simulink model "commhdlQPSKTxRx"  (R2025b)
settings: Solver=FixedStepDiscrete  StartTime=0.0  StopTime=stopTime  RelTol=1e-3
PostLoadFcn:
  | hScopeConfig = get_param([gcs '/Receiver/QPSK Rx/Frequency and Time Synchronizer/Symbol Synchronizer/No HDL/QPSK Receiver Eye Diagram'],'ScopeConfiguration');
  | 
  | hScopeConfig.OpenAtSimulationStart = false;
  | hScopeConfig.Visible = false;
  | SamplesPerSymbol = 4;
  | %UpsamplesRx = 1;
  | clear hScopeConfig
InitFcn:
  | commhdlQPSKTxRxModelInit;
  | % Rate bridge: ADRV9002/Jupiter radio runs at 15.36 MHz = 2x the 7.68 MHz
  | % (4 samples/symbol @ Rsym=1.92 MHz) the QPSK Rx requires. The deployed
  | % Receiver must downsample the ADC stream by 2. UpsamplesRx=1 fed the QPSK
  | % Rx 8 sps (2x-upsampled) and broke symbol sync / the loopback bit check.
  | UpsamplesRx = 1;   %% T8 RATE FIX: rail 15.36e6 == ADC bus rate,
  | %% no ingress decimation (was 2 when the rail sat on the 7.68e6 rung)
  | UpsamplesTx = 1;
  | clear simTimingOffset;
StopFcn:
  | if exist('simTimingOffset','var')
  |   disp('Simulation completed');
  |   %QPSKTxRxVerification;
  | end
undefined symbols (not defined in the file or in its folder): Add, Config, fsym, randsrc, RandStream, Rsym, Shift
libraries: hdlsllib x76, simulink x21, dspsigops x19, dsphdlfiltering2 x3, dsphdlsigops2 x2, dsphdlmathfun2 x2, commdigbbndpm3 x2, commchan3 x1, commrflib2 x1
(part 3 of 4)

== system commhdlQPSKTxRx/Receiver/QPSK Rx/Frequency and Time Synchronizer/Phase Ambiguity Estimation and Correction/Phase Ambiguity Estimator ==
  dataIn : Inport
  syncPulse : Inport  Port=2
  validIn : Inport  Port=3
  Compare To Constant : simulink/Logic and Bit Operations/Compare To Constant  relop===  const=7  OutDataTypeStr=boolean
  Delay{1..3,8} (4 alike) : Delay  DelayLength=1
  Delay{4..7,9..11} (7 alike) : Delay
  Direct Lookup Table (n-D) : LookupNDDirect  NumberOfTableDimensions=1  Table=fi(preambleSymbols(3+1:3+8),1,16)  DiagnosticForOutOfRangeInput=Error
  HDL Counter : hdlsllib/Sources/HDL Counter  CountType=Count limited  CountInit=0  CountStep=1  CountMax=8-1  CountFromType=Initial value  CountFrom=0  CountResetPort=on  CountLoadPort=off  CountEnbPort=on  CountDirPort=off  CountHitOutputPort=off  CountDataType=Unsigned  CountWordLen=3  CountFracLen=0  CountSampTime=1
  Logical Operator : Logic  IconShape=distinctive  AllPortsSameDT=off  OutDataTypeStr=boolean
  Math Function : Math  Operator=conj  SignedPower=on  RndMeth=Zero
  Product : Product
  Subsystem : Subsystem
  Subsystem1 : Subsystem
  endOut : Outport
  estOut : Outport  Port=2
  validOut : Outport  Port=3
  wires:
  Compare To Constant/1 -> Logical Operator/2
  Subsystem/1(Out2) -> Subsystem1/1(In1), HDL Counter/1
  Direct Lookup Table (n-D)/1 -> Math Function/1
  Math Function/1 -> Delay4/1
  Product/1 -> Delay9/1
  Delay8/1 -> Direct Lookup Table (n-D)/1
  Delay1/1 -> Delay5/1
  Delay2/1 -> Delay6/1
  Delay3/1 -> Delay7/1
  Delay4/1 -> Product/2
  Delay5/1 -> Product/1
  Delay6/1 -> Delay10/1
  Delay7/1 -> Delay11/1
  Delay9/1 -> estOut/1
  Delay10/1 -> validOut/1
  Delay11/1 -> endOut/1
  dataIn/1 -> Delay1/1
  HDL Counter/1 -> Delay8/1, Compare To Constant/1
  Subsystem1/1(validOut) -> Delay2/1, Logical Operator/1, HDL Counter/2
  Logical Operator/1 -> Delay3/1, Subsystem/2(H)
  syncPulse/1 -> Subsystem/1(L)
  validIn/1 -> Subsystem1/2(validIn)

== system commhdlQPSKTxRx/Receiver/QPSK Rx/Frequency and Time Synchronizer/Preamble Detector/Correlator ==
  dataIn : Inport
  validIn : Inport  Port=2
  Complex to Real-Imag : ComplexToRealImag  Output=Real
  Delay{1..6} (6 alike) : Delay  DelayLength=1
  Delay7 : Delay  DelayLength=4
  Delay8 : Delay  DelayLength=4
  Discrete FIR Filter : dsphdlfiltering2/Discrete FIR Filter  NumeratorSource=Property  Numerator=rxPreambleMFCoeffs  NumeratorPrototype=[]  FilterStructure=Direct form systolic  SerializationOption=Minimum number of cycles between valid input samples  NumCycles=2  NumberOfMultipliers=2  SimulateUsing=Code generation  roundingMode=Floor  overflowMode=off  CoefficientsDataTypeStr=Inherit: Same word length as input  OutputDataTypeStr=Inherit: Same word length as input  ResetInputPort=off  HDLGlobalReset=off  CoeffMultiplier=Multiplier  UseMultForPow2Coeff=on  FrameInputSymmOptim=off
  Magnitude Squared : Subsystem
  Magnitude Squared and Moving Sum : Subsystem
  ThresholdLimiter : MATLAB Function  TreatAsAtomicUnit=on
  dataOut : Outport
  threshold : Outport  Port=2
  validOut : Outport  Port=3
  wires:
  Discrete FIR Filter/2 -> Delay1/1
  validIn/1 -> Magnitude Squared and Moving Sum/2(validIn), Discrete FIR Filter/2
  Discrete FIR Filter/1 -> Delay6/1
  Delay1/1 -> Delay7/1
  Delay3/1 -> validOut/1
  dataIn/1 -> Magnitude Squared and Moving Sum/1(scaled1), Discrete FIR Filter/1
  Delay4/1 -> ThresholdLimiter/1(x)
  Delay2/1 -> dataOut/1
  Delay5/1 -> threshold/1
  Magnitude Squared and Moving Sum/1(E1) -> Delay4/1
  Delay6/1 -> Magnitude Squared/1(In1)
  Magnitude Squared/1(Out1) -> Complex to Real-Imag/1
  ThresholdLimiter/1(y) -> Delay8/1
  Delay7/1 -> Delay3/1
  Delay8/1 -> Delay5/1
  Complex to Real-Imag/1 -> Delay2/1

== system commhdlQPSKTxRx/Receiver/QPSK Rx/Frequency and Time Synchronizer/Preamble Detector/FIFO ==
  in : Inport
  push : Inport  Port=2
  pop : Inport  Port=3
  reset : Inport  Port=4
  Delay1 : Delay  DelayLength=1
  Pop Counter : hdlsllib/Sources/HDL Counter  CountType=Count limited  CountInit=0  CountStep=1  CountMax=fifoSize -1  CountFromType=Initial value  CountFrom=0  CountResetPort=on  CountLoadPort=off  CountEnbPort=on  CountDirPort=off  CountHitOutputPort=off  CountDataType=Unsigned  CountWordLen=nextpow2(fifoSize)  CountFracLen=0  CountSampTime=1
  Push Counter : hdlsllib/Sources/HDL Counter  CountType=Count limited  CountInit=0  CountStep=1  CountMax=fifoSize -1  CountFromType=Initial value  CountFrom=0  CountResetPort=on  CountLoadPort=off  CountEnbPort=on  CountDirPort=off  CountHitOutputPort=off  CountDataType=Unsigned  CountWordLen=nextpow2(fifoSize)  CountFracLen=0  CountSampTime=1
  Simple Dual Port RAM : hdlsllib/HDL RAMs/Simple Dual Port RAM  ram_size=nextpow2(fifoSize)
  Validate Input Push Pop : Subsystem
  out : Outport
  numEntries : Outport  Port=2
  validPop : Outport  Port=3
  wires:
  Delay1/1 -> Push Counter/1, Pop Counter/1
  in/1 -> Simple Dual Port RAM/1
  reset/1 -> Validate Input Push Pop/1(rst), Delay1/1
  Validate Input Push Pop/2(valid pop) -> Pop Counter/2, validPop/1
  Validate Input Push Pop/1(valid push) -> Push Counter/2, Simple Dual Port RAM/3
  pop/1 -> Validate Input Push Pop/3(pop)
  push/1 -> Validate Input Push Pop/2(push)
  Pop Counter/1 -> Simple Dual Port RAM/4
  Push Counter/1 -> Simple Dual Port RAM/2
  Simple Dual Port RAM/1 -> out/1
  Validate Input Push Pop/3(numEntries) -> numEntries/1

== system commhdlQPSKTxRx/Receiver/QPSK Rx/Frequency and Time Synchronizer/Preamble Detector/No HDL ==
  In1 : Inport
  In2 : Inport  Port=2
  Enable : EnablePort
  Correlation Time Scope : Scope  NumInputPorts=2
      settings: TimeUnits=Metric (based on Time Span)  Title=Time Plot of Preamble Detection  ActiveDisplayYMinimum=-0.38501295493915666  ActiveDisplayYMaximum=3.4651165944524109  YLabel=Amplitude
  Data Type Conversion : DataTypeConversion  OutDataTypeStr=double  SaturateOnIntegerOverflow=off  RndMeth=Floor
  Data Type Conversion1 : DataTypeConversion  OutDataTypeStr=double  SaturateOnIntegerOverflow=off  RndMeth=Floor
  To Workspace : ToWorkspace  VariableName=simPeakFind  SampleTime=-1
      settings: Save2DSignal=2-D array (concatenate along first dimension)
  wires:
  Data Type Conversion1/1 -> Correlation Time Scope/2  "Threshold"
  In2/1 -> Data Type Conversion1/1
  Data Type Conversion/1 -> To Workspace/1, Correlation Time Scope/1  "Correlation Value"
  In1/1 -> Data Type Conversion/1

== system commhdlQPSKTxRx/Receiver/QPSK Rx/Frequency and Time Synchronizer/Preamble Detector/Peak Search ==
  note: peak picker
  corr : Inport
  thresholdExceeded : Inport  Port=2
  validIn : Inport  Port=3
  Compare To Constant : simulink/Logic and Bit Operations/Compare To Constant  relop===  const=samplesPerFrame1x - 1  OutDataTypeStr=boolean
  Logical Operator : Logic  IconShape=distinctive  AllPortsSameDT=off  OutDataTypeStr=boolean
  Logical Operator4 : Logic  IconShape=distinctive  AllPortsSameDT=off  OutDataTypeStr=boolean
  Relational Operator : RelationalOperator  Operator=>  OutDataTypeStr=boolean  InputSameDT=off
  Terminator : Terminator
  Unit Delay Enabled Synchronous : hdlsllib/Discrete/Unit Delay Enabled Synchronous  InitialCondition=0.0  SampleTime=-1
  Unit Delay Enabled Synchronous1 : hdlsllib/Discrete/Unit Delay Enabled Synchronous  InitialCondition=0.0  SampleTime=-1
  Unit Delay Enabled Resettable Synchronous : hdlsllib/Discrete/Unit Delay Enabled Resettable Synchronous  InitialCondition=0.0  SampleTime=-1
  Unit Delay Enabled Resettable Synchronous1 : hdlsllib/Discrete/Unit Delay Enabled Resettable Synchronous  InitialCondition=0.0  SampleTime=-1
  timing Reference : hdlsllib/Sources/HDL Counter  CountType=Count limited  CountInit=0  CountStep=1  CountMax=samplesPerFrame1x - 1  CountFromType=Initial value  CountFrom=0  CountResetPort=off  CountLoadPort=off  CountEnbPort=on  CountDirPort=off  CountHitOutputPort=off  CountDataType=Unsigned  CountWordLen=nextpow2(samplesPerFrame1x - 1)  CountFracLen=0  CountSampTime=1
  timing Reference Long : hdlsllib/Sources/HDL Counter  CountType=Free running  CountInit=0  CountStep=1  CountMax=samplesPerFrame1x - 1  CountFromType=Initial value  CountFrom=0  CountResetPort=off  CountLoadPort=off  CountEnbPort=on  CountDirPort=off  CountHitOutputPort=off  CountDataType=Unsigned  CountWordLen=32  CountFracLen=0  CountSampTime=1
  timingOffset : Outport
  done : Outport  Port=2
  success : Outport  Port=3
  wires:
  validIn/1 -> Logical Operator/1, timing Reference/1, timing Reference Long/1
  timing Reference Long/1 -> Unit Delay Enabled Synchronous1/1
  timing Reference/1 -> Unit Delay Enabled Synchronous/1, Compare To Constant/1
  thresholdExceeded/1 -> Unit Delay Enabled Resettable Synchronous1/2, Unit Delay Enabled Resettable Synchronous1/1, Logical Operator4/2
  corr/1 -> Unit Delay Enabled Resettable Synchronous/1, Relational Operator/1
  Compare To Constant/1 -> Logical Operator/2
  Logical Operator/1 -> Unit Delay Enabled Resettable Synchronous1/3, done/1, Unit Delay Enabled Resettable Synchronous/3
  Relational Operator/1 -> Logical Operator4/1
  Unit Delay Enabled Resettable Synchronous/1 -> Relational Operator/2
  Unit Delay Enabled Resettable Synchronous1/1 -> success/1
  Logical Operator4/1 -> Unit Delay Enabled Synchronous/2, Unit Delay Enabled Synchronous1/2, Unit Delay Enabled Resettable Synchronous/2
  Unit Delay Enabled Synchronous/1 -> timingOffset/1
  Unit Delay Enabled Synchronous1/1 -> Terminator/1

== system commhdlQPSKTxRx/Receiver/QPSK Rx/Frequency and Time Synchronizer/Preamble Detector/Timing Adjust ==
  timingOffset : Inport
  timingOffsetValid : Inport  Port=2
  dataIn : Inport  Port=3
  validIn : Inport  Port=4
  Delay{,1..4} (5 alike) : Delay  DelayLength=1
  Logical Operator : Logic  AllPortsSameDT=off  OutDataTypeStr=boolean
  Logical Operator1 : Logic  Operator=NOT  AllPortsSameDT=off  OutDataTypeStr=boolean
  Logical Operator2 : Logic  Inputs=3  AllPortsSameDT=off  OutDataTypeStr=boolean
  No HDL : Subsystem
  Relational Operator : RelationalOperator  Operator===  OutDataTypeStr=boolean  InputSameDT=off
  State Register : hdlsllib/Discrete/Unit Delay Enabled Resettable Synchronous  InitialCondition=0.0  SampleTime=-1
  Unit Delay Enabled Synchronous3 : hdlsllib/Discrete/Unit Delay Enabled Synchronous  InitialCondition=0.0  SampleTime=-1
  timing Reference : hdlsllib/Sources/HDL Counter  CountType=Count limited  CountInit=0  CountStep=1  CountMax=searchSamples - 1  CountFromType=Initial value  CountFrom=0  CountResetPort=off  CountLoadPort=off  CountEnbPort=on  CountDirPort=off  CountHitOutputPort=off  CountDataType=Unsigned  CountWordLen=nextpow2(searchSamples - 1)  CountFracLen=0  CountSampTime=1
  dataOut : Outport
  validOut : Outport  Port=2
  SyncPulse : Outport  Port=3
  wires:
  Delay4/1 -> dataOut/1
  Delay3/1 -> validOut/1
  timingOffset/1 -> Unit Delay Enabled Synchronous3/1
  Unit Delay Enabled Synchronous3/1 -> Relational Operator/2
  Delay/1 -> SyncPulse/1
  validIn/1 -> timing Reference/1, Logical Operator2/1, No HDL/1(validIn), Delay3/1
  State Register/1 -> Logical Operator2/3, Delay1/1
  Logical Operator1/1 -> Logical Operator/2
  Relational Operator/1 -> Logical Operator2/2
  Logical Operator2/1 -> No HDL/3(syncPulse), Delay/1, Delay2/1
  Delay2/1 -> State Register/3
  Logical Operator/1 -> State Register/1, State Register/2, Unit Delay Enabled Synchronous3/2
  timing Reference/1 -> No HDL/2(timingOffset), Relational Operator/1
  timingOffsetValid/1 -> Logical Operator/1
  Delay1/1 -> Logical Operator1/1
  dataIn/1 -> Delay4/1

== system commhdlQPSKTxRx/Receiver/QPSK Rx/Frequency and Time Synchronizer/Symbol Synchronizer/Gardner TED ==
  data : Inport
  strobe : Inport  Port=2
  Constant : Constant  Value=0  OutDataTypeStr=Inherit: Inherit via back propagation  SampleTime=1/(Rsym*SamplesPerSymbol)
  Delay10 : Delay  DelayLength=4
  GTED : Subsystem
  Switch : Switch  Criteria=u2 ~= 0  InputSameDT=off
  e : Outport  VectorParamsAs1DForOutWhenUnconnected=off
  wires:
  Constant/1 -> Switch/3
  Switch/1 -> e/1
  strobe/1 -> Delay10/1
  data/1 -> GTED/1(In1)
  GTED/1(Out1) -> Switch/1
  Delay10/1 -> Switch/2

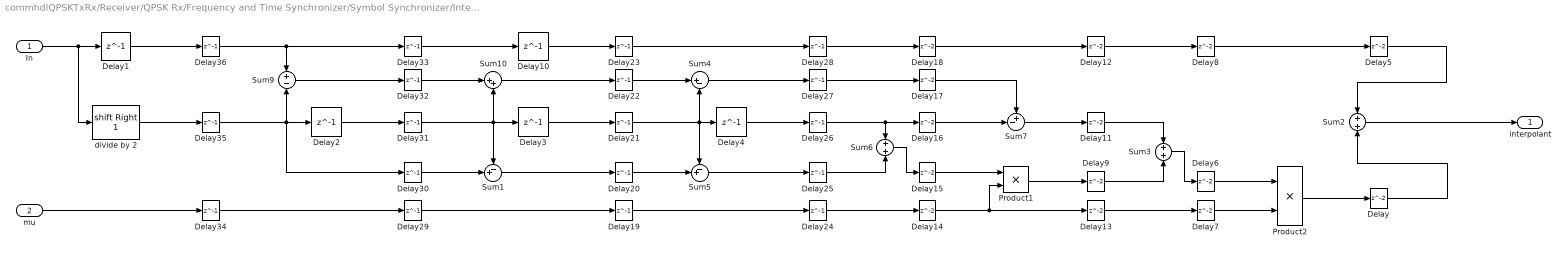
== system commhdlQPSKTxRx/Receiver/QPSK Rx/Frequency and Time Synchronizer/Symbol Synchronizer/Interpolation Filter ==
  In : Inport
  mu : Inport  Port=2
  Delay{,5..9,11..18} (14 alike) : Delay
  Delay{1..4,10} (5 alike) : Delay  DelayLength=1  InitialCondition=0
  Delay{19..36} (18 alike) : Delay  DelayLength=1
  Product1 : Product  OutDataTypeStr=fixdt(1,16,10)  RndMeth=Zero
  Product2 : Product  RndMeth=Zero  OutDataTypeStr=Inherit: Same as first input
  Sum1 : Sum  Inputs=-+|
  Sum10 : Sum  Inputs=|++
  Sum2 : Sum  Inputs=+|+
  Sum3 : Sum  Inputs=+|+  OutDataTypeStr=fixdt(1,16,10)
  Sum4 : Sum  Inputs=|+-
  Sum5 : Sum  Inputs=-+|
  Sum6 : Sum  Inputs=+|+  OutDataTypeStr=fixdt(1,16,11)  SaturateOnIntegerOverflow=on
  Sum7 : Sum  Inputs=+-|  OutDataTypeStr=fixdt(1,16,10)
  Sum9 : Sum  Inputs=+-
  divide by 2 : ArithShift  BitShiftNumber=1  BitShiftDirection=Right
  interpolant : Outport
  wires:
  Sum9/1 -> Delay32/1
  In/1 -> divide by 2/1, Delay1/1
  Sum2/1 -> interpolant/1
  Sum7/1 -> Delay11/1
  Product1/1 -> Delay9/1
  Product2/1 -> Delay/1
  Sum3/1 -> Delay6/1
  Sum1/1 -> Delay20/1
  Delay3/1 -> Delay21/1
  Sum10/1 -> Delay22/1
  Delay2/1 -> Delay31/1
  Delay1/1 -> Delay36/1
  divide by 2/1 -> Delay35/1
  Delay/1 -> Sum2/2
  Delay5/1 -> Sum2/1
  Delay6/1 -> Product2/1
  Delay7/1 -> Product2/2
  Delay8/1 -> Delay5/1
  Delay9/1 -> Sum3/2
  Delay11/1 -> Sum3/1
  Delay12/1 -> Delay8/1
  Delay13/1 -> Delay7/1
  Delay14/1 -> Delay13/1, Product1/2
  Delay15/1 -> Product1/1
  Delay16/1 -> Sum7/2
  Delay17/1 -> Sum7/1
  Delay18/1 -> Delay12/1
  mu/1 -> Delay34/1
  Sum5/1 -> Delay25/1
  Delay4/1 -> Delay26/1
  Sum4/1 -> Delay27/1
  Delay10/1 -> Delay23/1
  Delay24/1 -> Delay14/1
  Sum6/1 -> Delay15/1
  Delay26/1 -> Delay16/1, Sum6/1
  Delay27/1 -> Delay17/1
  Delay28/1 -> Delay18/1
  Delay25/1 -> Sum6/2
  Delay19/1 -> Delay24/1
  Delay20/1 -> Sum5/2
  Delay21/1 -> Sum4/2, Sum5/1, Delay4/1
  Delay22/1 -> Sum4/1
  Delay23/1 -> Delay28/1
  Delay29/1 -> Delay19/1
  Delay30/1 -> Sum1/2
  Delay31/1 -> Sum1/1, Sum10/2, Delay3/1
  Delay32/1 -> Sum10/1
  Delay33/1 -> Delay10/1
  Delay34/1 -> Delay29/1
  Delay35/1 -> Delay30/1, Delay2/1, Sum9/2
  Delay36/1 -> Delay33/1, Sum9/1

== system commhdlQPSKTxRx/Receiver/QPSK Rx/Frequency and Time Synchronizer/Symbol Synchronizer/Loop Filter ==
  note: Proportional-Plus-Integrator Loop Filter,
      | Infinite DC Response to guarantee convergence
  e : Inport
  Add : Sum
  Add2 : Sum  Inputs=|++  OutDataTypeStr=Inherit: Same as first input
  Data Type Conversion17 : DataTypeConversion  OutDataTypeStr=fixdt(1,11,10)  RndMeth=Floor
  Delay : Delay  DelayLength=1
  Delay1 : Delay  DelayLength=1  InitialCondition=0
  Delay2 : Delay  InitialCondition=0
  Delay3 : Delay  InitialCondition=0
  Delay4 : Delay  DelayLength=1  InitialCondition=0
  Delay5 : Delay  InitialCondition=0
  Delay6 : Delay  DelayLength=1
  IntegClamp : Saturate  UpperLimit=0.06  LowerLimit=-0.06
  K1 : Gain  Gain=fi(SSLoopFilterPropGain,1,24,24)  ParamDataTypeStr=Inherit: Inherit from 'Gain'  OutDataTypeStr=fixdt(1,30,23)
  K2 : Gain  Gain=fi(SSLoopFilterIntegGain,1,24,24)  ParamDataTypeStr=Inherit: Inherit from 'Gain'  OutDataTypeStr=fixdt(1,30,23)
  v : Outport
  wires:
  Delay/1 -> Add2/2
  Delay5/1 -> Delay6/1
  Delay3/1 -> Delay1/1
  e/1 -> Delay2/1
  Add/1 -> Data Type Conversion17/1
  Delay1/1 -> Add/1
  Delay4/1 -> Add/2
  Delay2/1 -> K1/1, K2/1
  Data Type Conversion17/1 -> v/1
  K2/1 -> Delay5/1
  K1/1 -> Delay3/1
  Delay6/1 -> Add2/1
  Add2/1 -> IntegClamp/1
  IntegClamp/1 -> Delay/1, Delay4/1

== system commhdlQPSKTxRx/Receiver/QPSK Rx/Frequency and Time Synchronizer/Symbol Synchronizer/No HDL ==
  data : Inport
  valid : Inport  Port=2
  Data Type Conversion : DataTypeConversion  OutDataTypeStr=double  SaturateOnIntegerOverflow=off  RndMeth=Floor
  No HDL : Subsystem
  QPSK Receiver Eye Diagram : EyeDiagramBlock  WindowPosition=[403.000000,370.000000,417.000000,506.000000,]  ScopeFrameLocation=window  SamplesPerSymbol=SamplesPerSymbol  SymbolsPerTrace=1  Title=RRC Matched Filtered Output  YLimits=[-1.1602,1.2629]
      settings: OpenAtSimulationStart=off
  Unit Delay Enabled Synchronous : hdlsllib/Discrete/Unit Delay Enabled Synchronous  InitialCondition=0.0  SampleTime=-1
  wires:
  data/1 -> No HDL/1(data), Unit Delay Enabled Synchronous/1
  Unit Delay Enabled Synchronous/1 -> Data Type Conversion/1
  valid/1 -> Unit Delay Enabled Synchronous/2, No HDL/Enable
  Data Type Conversion/1 -> QPSK Receiver Eye Diagram/1

== system commhdlQPSKTxRx/Receiver/QPSK Rx/Frequency and Time Synchronizer/Symbol Synchronizer/Rate Handle ==
  dataIn : Inport
  strobe : Inport  Port=2
  validIn : Inport  Port=3
  Compare To Constant : simulink/Logic and Bit Operations/Compare To Constant  relop===  const=0  OutDataTypeStr=boolean
  Constant : Constant  Value=false  SampleTime=-1
  FIFO : Subsystem  mask{fifoSize=32, pushFullDiag=Error, popEmptyDiag=Ignore}
      mask prompts: fifoSize "FIFO size:"; pushFullDiag "Push full FIFO:"; popEmptyDiag "Pop empty FIFO:"
      mask TypeOptions pushFullDiag: Ignore | Warning | Error
      mask TypeOptions popEmptyDiag: Ignore | Warning | Error
  HDL Counter : hdlsllib/Sources/HDL Counter  CountType=Count limited  CountInit=0  CountStep=1  CountMax=SamplesPerSymbol - 1  CountFromType=Initial value  CountFrom=0  CountResetPort=off  CountLoadPort=off  CountEnbPort=on  CountDirPort=off  CountHitOutputPort=off  CountDataType=Unsigned  CountWordLen=nextpow2(SamplesPerSymbol - 1)  CountFracLen=0  CountSampTime=1
  Logical Operator : Logic  AllPortsSameDT=off  OutDataTypeStr=boolean
  Terminator : Terminator
  dataOut : Outport
  validOut : Outport  Port=2
  wires:
  strobe/1 -> FIFO/2(push)
  dataIn/1 -> FIFO/1(in)
  validIn/1 -> Logical Operator/1, HDL Counter/1
  HDL Counter/1 -> Compare To Constant/1
  Compare To Constant/1 -> Logical Operator/2
  Logical Operator/1 -> FIFO/3(pop)
  FIFO/1(out) -> dataOut/1
  FIFO/3(validPop) -> validOut/1
  FIFO/2(numEntries) -> Terminator/1
  Constant/1 -> FIFO/4(reset)

== system commhdlQPSKTxRx/Transmitter/QPSK Tx/Bit Packetizer/Data Bits FIFO/No HDL ==
  push : Inport
  pop : Inport  Port=2
  MATLAB Function : MATLAB Function  TreatAsAtomicUnit=on
  No HDL : Subsystem
  wires:
  push/1 -> MATLAB Function/1(wr), No HDL/1(push)
  pop/1 -> MATLAB Function/2(rd), No HDL/5(pop)
  MATLAB Function/2(ncount) -> No HDL/3(ncount)
  MATLAB Function/1(full) -> No HDL/2(full)
  MATLAB Function/3(empty) -> No HDL/4(empty)

== system commhdlQPSKTxRx/Transmitter/QPSK Tx/Bit Packetizer/Preamble Bits Generator/Preamble Bits Store ==
  note: The Preamble is padded with zeros in the LUT such that
      | the length is the 2^nextpow2(length(Preamble)) for
      | efficient resource mapping to RAM
  actualPreamble : Inport
  sampleCount : Inport  Port=2
  Constant : Constant  OutDataTypeStr=boolean  SampleTime=1/(Rsym*SamplesPerSymbol)
  Extract Bits : simulink/Logic and Bit Operations/Extract Bits  bitsToExtract=Range of bits  numBits=8  bitIdxRange=[0 nextpow2(length(Preamble))-1]  outScalingMode=Treat bit field as an integer
  Preamble : LookupNDDirect  NumberOfTableDimensions=1  Table=[Preamble;false(32-length(Preamble),1)]  DiagnosticForOutOfRangeInput=Error
  Switch : Switch  Criteria=u2 ~= 0  Threshold=1  SaturateOnIntegerOverflow=off  InputSameDT=off
  preamble : Outport
  wires:
  Switch/1 -> preamble/1
  Constant/1 -> Switch/3
  Extract Bits/1 -> Preamble/1
  Preamble/1 -> Switch/1
  sampleCount/1 -> Extract Bits/1
  actualPreamble/1 -> Switch/2

== system commhdlQPSKTxRx/Receiver/QPSK Rx/Frequency and Time Synchronizer/Coarse Frequency Compensator/Coarse Frequency Estimator/Extract Frequency ==
  datain : Inport
  validIn : Inport  Port=2
  Complex to Magnitude-Angle HDL Optimized : dsphdlmathfun2/Complex to Magnitude-Angle  NumIterationsSource=Auto  NumIterations=10  OutputFormat=Angle  AngleFormat=Normalized  ScaleOutput=on  ScalingMethod=Shift-Add  SimulateUsing=Code generation
  Delay{1..4} (4 alike) : Delay  DelayLength=1
  Gain : Gain  Gain=1/2  ParamDataTypeStr=fixdt(0,1,1)  OutDataTypeStr=Inherit: Same as input
  Unit Delay Enabled Synchronous : hdlsllib/Discrete/Unit Delay Enabled Synchronous  InitialCondition=0.0  SampleTime=-1
  normFreqOut : Outport
  wires:
  Unit Delay Enabled Synchronous/1 -> Delay2/1
  Complex to Magnitude-Angle HDL Optimized/2 -> Unit Delay Enabled Synchronous/2
  datain/1 -> Delay1/1
  Gain/1 -> Delay3/1
  Delay1/1 -> Complex to Magnitude-Angle HDL Optimized/1
  Delay2/1 -> Gain/1
  Delay3/1 -> normFreqOut/1
  validIn/1 -> Delay4/1
  Delay4/1 -> Complex to Magnitude-Angle HDL Optimized/2
  Complex to Magnitude-Angle HDL Optimized/1 -> Unit Delay Enabled Synchronous/1

== system commhdlQPSKTxRx/Receiver/QPSK Rx/Frequency and Time Synchronizer/Coarse Frequency Compensator/Coarse Frequency Estimator/Integrator ==
  note: store the value in the Reg before reset
  dataIn : Inport
  validIn : Inport  Port=2
  Add1 : Sum  Inputs=|++  OutDataTypeStr=Inherit: Same as first input
  Delay : Delay  DelayLength=1
  Delay1 : Delay  DelayLength=1
  Delay2 : Delay  DelayLength=1
  Integ Reg : hdlsllib/Discrete/Unit Delay Enabled Resettable Synchronous  InitialCondition=0.0  SampleTime=-1
  Reset Generator : Subsystem
  Store Reg : hdlsllib/Discrete/Unit Delay Enabled Synchronous  InitialCondition=0.0  SampleTime=-1
  IntegOut : Outport
  IntegValid : Outport  Port=2
  wires:
  Add1/1 -> Integ Reg/1
  Integ Reg/1 -> Store Reg/1, Add1/2
  validIn/1 -> Delay2/1, Reset Generator/1(validIn)
  dataIn/1 -> Delay1/1
  Delay1/1 -> Add1/1
  Delay/1 -> IntegValid/1
  Store Reg/1 -> IntegOut/1
  Reset Generator/1(reset) -> Delay/1, Store Reg/2, Integ Reg/3
  Delay2/1 -> Integ Reg/2

== system commhdlQPSKTxRx/Receiver/QPSK Rx/Frequency and Time Synchronizer/Phase Ambiguity Estimation and Correction/Phase Ambiguity Corrector/Reciprocal ==
  dataIn : Inport
  Compare To Constant : simulink/Logic and Bit Operations/Compare To Constant  relop=<  const=0  OutDataTypeStr=boolean
  Data Type Conversion : DataTypeConversion  OutDataTypeStr=fixdt(1,WL,0)  ConvertRealWorld=Stored Integer (SI)  SaturateOnIntegerOverflow=off  RndMeth=Floor
  Data Type Conversion1 : DataTypeConversion  OutDataTypeStr=fixdt(0,LUTAddrWL,0)  ConvertRealWorld=Stored Integer (SI)  SaturateOnIntegerOverflow=off  RndMeth=Floor
  Data Type Conversion2 : DataTypeConversion  OutDataTypeStr=fixdt(0,WL-LUTAddrWL,0)  ConvertRealWorld=Stored Integer (SI)  SaturateOnIntegerOverflow=off  RndMeth=Floor
  Delay : Delay  DelayLength=1
  Delay1 : Delay  DelayLength=1
  Delay2 : Delay  DelayLength=1
  Extract Bits : simulink/Logic and Bit Operations/Extract Bits  bitsToExtract=Range ending with least significant bit  numBits=LUTAddrWL  bitIdxRange=[0 7]  outScalingMode=Treat bit field as an integer
  Function Impl : Subsystem
  dataOut : Outport
  wires:
  dataIn/1 -> Data Type Conversion/1
  Extract Bits/1 -> Delay2/1
  Data Type Conversion/1 -> Delay/1
  Compare To Constant/1 -> Delay1/1
  Data Type Conversion1/1 -> Function Impl/2(LUTAddr)
  Function Impl/1(functionValues) -> dataOut/1
  Delay/1 -> Compare To Constant/1, Extract Bits/1
  Delay1/1 -> Data Type Conversion2/1
  Delay2/1 -> Data Type Conversion1/1
  Data Type Conversion2/1 -> Function Impl/1(switch)

== system commhdlQPSKTxRx/Receiver/QPSK Rx/Frequency and Time Synchronizer/Phase Ambiguity Estimation and Correction/Phase Ambiguity Estimator/Subsystem ==
  L : Inport
  H : Inport  Port=2
  Delay6 : Delay  DelayLength=1  InitialCondition=1
  Logical Operator : Logic  AllPortsSameDT=off  OutDataTypeStr=boolean
  Logical Operator1 : Logic  Operator=NOT  IconShape=distinctive  AllPortsSameDT=off  OutDataTypeStr=boolean
  Logical Operator2 : Logic  Operator=OR  AllPortsSameDT=off  OutDataTypeStr=boolean
  Out2 : Outport
  wires:
  L/1 -> Logical Operator1/1
  H/1 -> Logical Operator2/1
  Delay6/1 -> Out2/1, Logical Operator/2
  Logical Operator1/1 -> Logical Operator/1
  Logical Operator/1 -> Logical Operator2/2
  Logical Operator2/1 -> Delay6/1

== system commhdlQPSKTxRx/Receiver/QPSK Rx/Frequency and Time Synchronizer/Phase Ambiguity Estimation and Correction/Phase Ambiguity Estimator/Subsystem1 ==
  In1 : Inport
  validIn : Inport  Port=2
  Logical Operator1 : Logic  IconShape=distinctive  AllPortsSameDT=off  OutDataTypeStr=boolean
  Logical Operator2 : Logic  Operator=NOT  IconShape=distinctive  AllPortsSameDT=off  OutDataTypeStr=boolean
  validOut : Outport
  wires:
  In1/1 -> Logical Operator2/1
  validIn/1 -> Logical Operator1/2
  Logical Operator1/1 -> validOut/1
  Logical Operator2/1 -> Logical Operator1/1

== system commhdlQPSKTxRx/Receiver/QPSK Rx/Frequency and Time Synchronizer/Preamble Detector/Correlator/Magnitude Squared ==
  In1 : Inport
  Delay1 : Delay
  Delay2 : Delay
  Delay3 : Delay
  Math Function : Math  Operator=conj
  Product : Product
  Out1 : Outport
  wires:
  In1/1 -> Math Function/1, Delay2/1
  Math Function/1 -> Delay1/1
  Product/1 -> Delay3/1
  Delay2/1 -> Product/1
  Delay1/1 -> Product/2
  Delay3/1 -> Out1/1

== system commhdlQPSKTxRx/Receiver/QPSK Rx/Frequency and Time Synchronizer/Preamble Detector/Correlator/Magnitude Squared and Moving Sum ==
  scaled1 : Inport
  validIn : Inport  Port=2
  Add : Sum  Inputs=|+-  OutDataTypeStr=Inherit: Same as first input
  Add1 : Sum  Inputs=|++  OutDataTypeStr=Inherit: Same as first input
  Complex to Real-Imag1 : ComplexToRealImag  Output=Real
  Delay : Delay  DelayLength=13  ShowEnablePort=on
      settings: InputPortMap=u0,e6
  Delay{1..4,6,8..10,12} (9 alike) : Delay
  Delay11 : Delay  DelayLength=11
  Delay14 : Delay  DelayLength=1  ShowEnablePort=on
      settings: InputPortMap=u0,e6
  Delay5 : Delay  DelayLength=1
  Delay7 : Delay  DelayLength=1
  Gain : Gain  Gain=ThresoldGainFac  OutDataTypeStr=Inherit: Same as input
  Math Function1 : Math  Operator=conj
  Product1 : Product
  E1 : Outport
  wires:
  Add/1 -> Delay5/1
  validIn/1 -> Delay12/1
  Delay/1 -> Add/2
  Delay14/1 -> Add1/2
  Complex to Real-Imag1/1 -> Delay3/1
  Add1/1 -> Delay11/1, Delay14/1
  Delay11/1 -> E1/1
  scaled1/1 -> Delay6/1, Math Function1/1
  Math Function1/1 -> Delay1/1
  Product1/1 -> Delay2/1
  Gain/1 -> Delay4/1
  Delay6/1 -> Product1/1
  Delay1/1 -> Product1/2
  Delay2/1 -> Complex to Real-Imag1/1
  Delay3/1 -> Gain/1
  Delay4/1 -> Delay/1, Add/1
  Delay5/1 -> Add1/1
  Delay7/1 -> Delay14/2
  Delay8/1 -> Delay/2, Delay7/1
  Delay9/1 -> Delay8/1
  Delay10/1 -> Delay9/1
  Delay12/1 -> Delay10/1

== system commhdlQPSKTxRx/Receiver/QPSK Rx/Frequency and Time Synchronizer/Preamble Detector/FIFO/Validate Input Push Pop ==
  rst : Inport
  push : Inport  Port=2
  pop : Inport  Port=3
  Compare To Constant : hdlsllib/Logic and Bit Operations/Compare To Constant  relop===  const=0  OutDataTypeStr=boolean
  Compare To Constant1 : hdlsllib/Logic and Bit Operations/Compare To Constant  relop===  const=fifoSize  OutDataTypeStr=boolean
  Constant : Constant  Value=true  SampleTime=-1
  Constant1 : Constant  Value=false  SampleTime=-1
  Delay : Delay  DelayLength=1
  Logical Operator1 : Logic  Operator=XOR  AllPortsSameDT=off  OutDataTypeStr=boolean
  Logical Operator2 : Logic  Operator=NOT  AllPortsSameDT=off  OutDataTypeStr=boolean
  Logical Operator{3..5,7,9} (5 alike) : Logic  AllPortsSameDT=off  OutDataTypeStr=boolean
  Logical Operator6 : Logic  Operator=NOT  AllPortsSameDT=off  OutDataTypeStr=boolean
  Logical Operator8 : Logic  Operator=NOT  AllPortsSameDT=off  OutDataTypeStr=boolean
  MATLAB Function : MATLAB Function  TreatAsAtomicUnit=on  mask{initVal=0, countToVal=fifoSize}
      mask prompts: initVal "Initial value:"; countToVal "Count to value:"
  No HDL : Subsystem
  Switch : Switch  Criteria=u2 ~= 0  SaturateOnIntegerOverflow=off  InputSameDT=off
  valid push : Outport
  valid pop : Outport  Port=2
  numEntries : Outport  Port=3
  wires:
  Logical Operator9/1 -> Logical Operator1/1, valid push/1
  Logical Operator2/1 -> Logical Operator9/2
  Logical Operator5/1 -> Logical Operator4/1
  Logical Operator8/1 -> Logical Operator5/2
  push/1 -> Logical Operator5/1, Logical Operator9/1
  Logical Operator1/1 -> MATLAB Function/2(enb)
  Logical Operator6/1 -> Logical Operator7/2
  Logical Operator7/1 -> Switch/2, valid pop/1, Logical Operator8/1, Logical Operator1/2
  Compare To Constant1/1 -> Logical Operator4/2
  Constant/1 -> Switch/3
  Logical Operator4/1 -> No HDL/1(pushFullFIFO), Logical Operator2/1  "push on full FIFO"
  Logical Operator3/1 -> No HDL/2(popEmptyFIFO), Logical Operator6/1  "pop on empty FIFO"
  Constant1/1 -> Switch/1
  MATLAB Function/1(count) -> Delay/1
  Switch/1 -> MATLAB Function/3(dir)
  pop/1 -> Logical Operator3/2, Logical Operator7/1
  Compare To Constant/1 -> Logical Operator3/1
  rst/1 -> MATLAB Function/1(rst)
  Delay/1 -> Compare To Constant1/1, numEntries/1, Compare To Constant/1

== system commhdlQPSKTxRx/Receiver/QPSK Rx/Frequency and Time Synchronizer/Preamble Detector/Timing Adjust/No HDL ==
  note: This subsystem generates variables required for QPSKRxVerification for validation
  validIn : Inport
  timingOffset : Inport  Port=2
  syncPulse : Inport  Port=3
  Compare To Constant : simulink/Logic and Bit Operations/Compare To Constant  relop===  const=0  OutDataTypeStr=boolean
  Delay : Delay  DelayLength=4
  Delay1 : Delay  DelayLength=4
  Frame Counter : hdlsllib/Sources/HDL Counter  CountType=Free running  CountInit=0  CountStep=1  CountMax=bitsPerPacket/2 - 1  CountFromType=Initial value  CountFrom=0  CountResetPort=off  CountLoadPort=off  CountEnbPort=on  CountDirPort=off  CountHitOutputPort=off  CountDataType=Unsigned  CountWordLen=32  CountFracLen=0  CountSampTime=1
  Logical Operator : Logic  AllPortsSameDT=off  OutDataTypeStr=boolean
  No HDL : Subsystem
  No HDL1 : Subsystem
  Symbol Counter : hdlsllib/Sources/HDL Counter  CountType=Count limited  CountInit=0  CountStep=1  CountMax=bitsPerPacket/2 - 1  CountFromType=Initial value  CountFrom=0  CountResetPort=off  CountLoadPort=off  CountEnbPort=on  CountDirPort=off  CountHitOutputPort=off  CountDataType=Unsigned  CountWordLen=nextpow2(bitsPerPacket/2 - 1)  CountFracLen=0  CountSampTime=1
  Unit Delay Enabled Synchronous : hdlsllib/Discrete/Unit Delay Enabled Synchronous  InitialCondition=0.0  SampleTime=-1
  wires:
  timingOffset/1 -> Delay1/1
  validIn/1 -> Logical Operator/2, Symbol Counter/1
  Symbol Counter/1 -> Compare To Constant/1
  Logical Operator/1 -> Unit Delay Enabled Synchronous/2, Frame Counter/1
  Compare To Constant/1 -> Logical Operator/1
  Frame Counter/1 -> Unit Delay Enabled Synchronous/1
  syncPulse/1 -> Delay/1
  Unit Delay Enabled Synchronous/1 -> No HDL1/1(frameNumber)
  Delay/1 -> No HDL/Enable, No HDL1/Enable
  Delay1/1 -> No HDL/1(timingOffset)

== system commhdlQPSKTxRx/Receiver/QPSK Rx/Frequency and Time Synchronizer/Symbol Synchronizer/Gardner TED/GTED ==
  In1 : Inport
  Add : Sum
  Add1 : Sum  Inputs=+-
  Add2 : Sum  Inputs=+-
  Complex to Real-Imag : ComplexToRealImag
  Delay{,1..7} (8 alike) : Delay  DelayLength=1
  Delay{8..13} (6 alike) : Delay
  Product : Product
  Product1 : Product
  Out1 : Outport
  wires:
  Product/1 -> Delay10/1
  Product1/1 -> Delay13/1
  Add/1 -> Out1/1
  In1/1 -> Complex to Real-Imag/1
  Complex to Real-Imag/1 -> Add1/2, Delay/1
  Delay3/1 -> Add1/1
  Delay/1 -> Delay1/1
  Delay2/1 -> Delay3/1
  Add1/1 -> Delay9/1
  Delay1/1 -> Delay2/1, Delay8/1
  Delay5/1 -> Delay11/1, Delay6/1
  Add2/1 -> Delay12/1
  Delay6/1 -> Delay7/1
  Delay4/1 -> Delay5/1
  Delay7/1 -> Add2/1
  Complex to Real-Imag/2 -> Add2/2, Delay4/1
  Delay8/1 -> Product/1
  Delay9/1 -> Product/2
  Delay10/1 -> Add/1
  Delay11/1 -> Product1/1
  Delay12/1 -> Product1/2
  Delay13/1 -> Add/2

== system commhdlQPSKTxRx/Receiver/QPSK Rx/Frequency and Time Synchronizer/Symbol Synchronizer/No HDL/No HDL ==
  data : Inport
  Enable : EnablePort
  Data Type Conversion : DataTypeConversion  OutDataTypeStr=double  SaturateOnIntegerOverflow=off  RndMeth=Floor
  QPSK Receiver Constellation 1 : ConstellationDiagram  WindowPosition=[436.000000,110.000000,915.000000,708.000000,]  Visible=on  ScopeFrameLocation=window  SymbolsToDisplaySource=Property  SymbolsToDisplay=10000  Title=Before Symbol Synchronization  XLimits=[-1.9386 1.9401]  YLimits=[-1.9386 1.9401]  AxesLimits=[-1.9386 1.9401]  DefaultConfigurationName=comm.scopes.ConstellationDiagramBlockCfg
      settings: OpenAtSimulationStart=off
  To Workspace : ToWorkspace  VariableName=simBeforeSS  SampleTime=-1
      settings: Save2DSignal=2-D array (concatenate along first dimension)
  wires:
  Data Type Conversion/1 -> To Workspace/1, QPSK Receiver Constellation 1/1
  data/1 -> Data Type Conversion/1

== system commhdlQPSKTxRx/Receiver/QPSK Rx/Frequency and Time Synchronizer/Symbol Synchronizer/Rate Handle/FIFO ==
  in : Inport
  push : Inport  Port=2
  pop : Inport  Port=3
  reset : Inport  Port=4
  Delay1 : Delay  DelayLength=1
  Pop Counter : hdlsllib/Sources/HDL Counter  CountType=Count limited  CountInit=0  CountStep=1  CountMax=fifoSize -1  CountFromType=Initial value  CountFrom=0  CountResetPort=on  CountLoadPort=off  CountEnbPort=on  CountDirPort=off  CountHitOutputPort=off  CountDataType=Unsigned  CountWordLen=nextpow2(fifoSize)  CountFracLen=0  CountSampTime=1
  Push Counter : hdlsllib/Sources/HDL Counter  CountType=Count limited  CountInit=0  CountStep=1  CountMax=fifoSize -1  CountFromType=Initial value  CountFrom=0  CountResetPort=on  CountLoadPort=off  CountEnbPort=on  CountDirPort=off  CountHitOutputPort=off  CountDataType=Unsigned  CountWordLen=nextpow2(fifoSize)  CountFracLen=0  CountSampTime=1
  Simple Dual Port RAM : hdlsllib/HDL RAMs/Simple Dual Port RAM  ram_size=nextpow2(fifoSize)
  Validate Input Push Pop : Subsystem
  out : Outport
  numEntries : Outport  Port=2
  validPop : Outport  Port=3
  wires:
  Delay1/1 -> Push Counter/1, Pop Counter/1
  in/1 -> Simple Dual Port RAM/1
  reset/1 -> Validate Input Push Pop/1(rst), Delay1/1
  Validate Input Push Pop/2(valid pop) -> Pop Counter/2, validPop/1
  Validate Input Push Pop/1(valid push) -> Push Counter/2, Simple Dual Port RAM/3
  pop/1 -> Validate Input Push Pop/3(pop)
  push/1 -> Validate Input Push Pop/2(push)
  Pop Counter/1 -> Simple Dual Port RAM/4
  Push Counter/1 -> Simple Dual Port RAM/2
  Simple Dual Port RAM/1 -> out/1
  Validate Input Push Pop/3(numEntries) -> numEntries/1

== system commhdlQPSKTxRx/Transmitter/QPSK Tx/Bit Packetizer/Data Bits FIFO/No HDL/No HDL ==
  push : Inport
  full : Inport  Port=2
  ncount : Inport  Port=3
  empty : Inport  Port=4
  pop : Inport  Port=5
  Assertion : Assertion
  Assertion1 : Assertion
  Display : Display
  Logical Operator : Logic  Operator=NAND  AllPortsSameDT=off  OutDataTypeStr=boolean
  Logical Operator1 : Logic  Operator=NAND  AllPortsSameDT=off  OutDataTypeStr=boolean
  wires:
  Logical Operator1/1 -> Assertion1/1
  ncount/1 -> Display/1
  Logical Operator/1 -> Assertion/1
  pop/1 -> Logical Operator1/2
  full/1 -> Logical Operator/2
  empty/1 -> Logical Operator1/1
  push/1 -> Logical Operator/1

== system commhdlQPSKTxRx/Receiver/QPSK Rx/Frequency and Time Synchronizer/Coarse Frequency Compensator/Coarse Frequency Estimator/Integrator/Reset Generator ==
  validIn : Inport
  Compare To Constant : simulink/Logic and Bit Operations/Compare To Constant  relop===  const=integAvgLen  OutDataTypeStr=boolean
  Delay1 : Delay  DelayLength=1
  Delay5 : Delay  DelayLength=1
  HDL Counter : hdlsllib/Sources/HDL Counter  CountType=Count limited  CountInit=0  CountStep=1  CountMax=integAvgLen  CountFromType=Initial value  CountFrom=0  CountResetPort=off  CountLoadPort=off  CountEnbPort=on  CountDirPort=off  CountHitOutputPort=off  CountDataType=Unsigned  CountWordLen=nextpow2(integAvgLen + 1)  CountFracLen=0  CountSampTime=1
  Logical Operator : Logic  AllPortsSameDT=off  OutDataTypeStr=boolean
  reset : Outport
  wires:
  Delay1/1 -> Logical Operator/1
  Delay5/1 -> Compare To Constant/1
  Logical Operator/1 -> reset/1
  validIn/1 -> HDL Counter/1, Delay1/1
  Compare To Constant/1 -> Logical Operator/2
  HDL Counter/1 -> Delay5/1

== system commhdlQPSKTxRx/Receiver/QPSK Rx/Frequency and Time Synchronizer/Phase Ambiguity Estimation and Correction/Phase Ambiguity Corrector/Reciprocal/Function Impl ==
  switch : Inport
  LUTAddr : Inport  Port=2
  Delay{6..8,10,15..16} (6 alike) : Delay
  Delay9 : Delay  DelayLength=1
  LUT1 : LookupNDDirect  NumberOfTableDimensions=1  Table=LUT(:,1)  DiagnosticForOutOfRangeInput=Error
  LUT2 : LookupNDDirect  NumberOfTableDimensions=1  Table=LUT(:,2)  DiagnosticForOutOfRangeInput=Error
  Multiport Switch : MultiPortSwitch  DataPortOrder=Zero-based contiguous  Inputs=2  zeroidx=on  SaturateOnIntegerOverflow=off  InputSameDT=off
  functionValues : Outport
  wires:
  Multiport Switch/1 -> Delay9/1
  Delay6/1 -> LUT1/1
  Delay7/1 -> LUT2/1
  Delay8/1 -> Delay10/1
  switch/1 -> Delay8/1
  LUT1/1 -> Delay16/1
  LUT2/1 -> Delay15/1
  Delay9/1 -> functionValues/1
  Delay10/1 -> Multiport Switch/1
  Delay16/1 -> Multiport Switch/3
  Delay15/1 -> Multiport Switch/2
  LUTAddr/1 -> Delay6/1, Delay7/1

== system commhdlQPSKTxRx/Receiver/QPSK Rx/Frequency and Time Synchronizer/Preamble Detector/FIFO/Validate Input Push Pop/No HDL ==
  pushFullFIFO : Inport
  popEmptyFIFO : Inport  Port=2
  Constant2 : Constant  Value=pushFullDiag  SampleTime=-1
  Constant3 : Constant  Value=popEmptyDiag  SampleTime=-1
  MATLAB Function : MATLAB Function  TreatAsAtomicUnit=on
  wires:
  Constant2/1 -> MATLAB Function/1(pushFullDiag)
  Constant3/1 -> MATLAB Function/2(popEmptyDiag)
  popEmptyFIFO/1 -> MATLAB Function/4(popEmpty)
  pushFullFIFO/1 -> MATLAB Function/3(pushFull)

== system commhdlQPSKTxRx/Receiver/QPSK Rx/Frequency and Time Synchronizer/Preamble Detector/Timing Adjust/No HDL/No HDL ==
  timingOffset : Inport
  Enable : EnablePort
  Data Type Conversion : DataTypeConversion  OutDataTypeStr=double  SaturateOnIntegerOverflow=off  RndMeth=Floor
  To Workspace : ToWorkspace  VariableName=simTimingOffset  SampleTime=-1
      settings: Save2DSignal=2-D array (concatenate along first dimension)
  wires:
  Data Type Conversion/1 -> To Workspace/1
  timingOffset/1 -> Data Type Conversion/1

== system commhdlQPSKTxRx/Receiver/QPSK Rx/Frequency and Time Synchronizer/Preamble Detector/Timing Adjust/No HDL/No HDL1 ==
  frameNumber : Inport
  Enable : EnablePort
  Data Type Conversion : DataTypeConversion  OutDataTypeStr=double  SaturateOnIntegerOverflow=off  RndMeth=Floor
  To Workspace : ToWorkspace  VariableName=simSyncedPackets  SampleTime=-1
      settings: Save2DSignal=2-D array (concatenate along first dimension)
  wires:
  frameNumber/1 -> Data Type Conversion/1
  Data Type Conversion/1 -> To Workspace/1

== system commhdlQPSKTxRx/Receiver/QPSK Rx/Frequency and Time Synchronizer/Symbol Synchronizer/Rate Handle/FIFO/Validate Input Push Pop ==
  rst : Inport
  push : Inport  Port=2
  pop : Inport  Port=3
  Compare To Constant : hdlsllib/Logic and Bit Operations/Compare To Constant  relop===  const=0  OutDataTypeStr=boolean
  Compare To Constant1 : hdlsllib/Logic and Bit Operations/Compare To Constant  relop===  const=fifoSize  OutDataTypeStr=boolean
  Constant : Constant  Value=true  SampleTime=-1
  Constant1 : Constant  Value=false  SampleTime=-1
  Delay : Delay  DelayLength=1
  Logical Operator1 : Logic  Operator=XOR  AllPortsSameDT=off  OutDataTypeStr=boolean
  Logical Operator2 : Logic  Operator=NOT  AllPortsSameDT=off  OutDataTypeStr=boolean
  Logical Operator{3..5,7,9} (5 alike) : Logic  AllPortsSameDT=off  OutDataTypeStr=boolean
  Logical Operator6 : Logic  Operator=NOT  AllPortsSameDT=off  OutDataTypeStr=boolean
  Logical Operator8 : Logic  Operator=NOT  AllPortsSameDT=off  OutDataTypeStr=boolean
  MATLAB Function : MATLAB Function  TreatAsAtomicUnit=on  mask{initVal=0, countToVal=fifoSize}
      mask prompts: initVal "Initial value:"; countToVal "Count to value:"
  No HDL : Subsystem
  Switch : Switch  Criteria=u2 ~= 0  SaturateOnIntegerOverflow=off  InputSameDT=off
  valid push : Outport
  valid pop : Outport  Port=2
  numEntries : Outport  Port=3
  wires:
  Logical Operator9/1 -> Logical Operator1/1, valid push/1
  Logical Operator2/1 -> Logical Operator9/2
  Logical Operator5/1 -> Logical Operator4/1
  Logical Operator8/1 -> Logical Operator5/2
  push/1 -> Logical Operator5/1, Logical Operator9/1
  Logical Operator1/1 -> MATLAB Function/2(enb)
  Logical Operator6/1 -> Logical Operator7/2
  Logical Operator7/1 -> Switch/2, valid pop/1, Logical Operator8/1, Logical Operator1/2
  Compare To Constant1/1 -> Logical Operator4/2
  Constant/1 -> Switch/3
  Logical Operator4/1 -> No HDL/1(pushFullFIFO), Logical Operator2/1  "push on full FIFO"
  Logical Operator3/1 -> No HDL/2(popEmptyFIFO), Logical Operator6/1  "pop on empty FIFO"
  Constant1/1 -> Switch/1
  MATLAB Function/1(count) -> Delay/1
  Switch/1 -> MATLAB Function/3(dir)
  pop/1 -> Logical Operator3/2, Logical Operator7/1
  Compare To Constant/1 -> Logical Operator3/1
  rst/1 -> MATLAB Function/1(rst)
  Delay/1 -> Compare To Constant1/1, numEntries/1, Compare To Constant/1

== system commhdlQPSKTxRx/Receiver/QPSK Rx/Frequency and Time Synchronizer/Symbol Synchronizer/Rate Handle/FIFO/Validate Input Push Pop/No HDL ==
  pushFullFIFO : Inport
  popEmptyFIFO : Inport  Port=2
  Constant2 : Constant  Value=pushFullDiag  SampleTime=-1
  Constant3 : Constant  Value=popEmptyDiag  SampleTime=-1
  MATLAB Function : MATLAB Function  TreatAsAtomicUnit=on
  wires:
  Constant2/1 -> MATLAB Function/1(pushFullDiag)
  Constant3/1 -> MATLAB Function/2(popEmptyDiag)
  popEmptyFIFO/1 -> MATLAB Function/4(popEmpty)
  pushFullFIFO/1 -> MATLAB Function/3(pushFull)

== matlab function commhdlQPSKTxRx/Receiver/Capture Data Bits/MATLAB Function ==
  data: valid input; datain input; start input; stop input; count_out output; packets_out output; bit_errors_out output
function [count_out, packets_out, bit_errors_out] = msgdec(valid, datain, start, stop)

persistent count;
persistent msgbuffer;

persistent packetsReceived
persistent errors;

if isempty(count) || isempty(msgbuffer) || isempty(packetsReceived)
    count = uint32(0);
    msgbuffer = zeros(1,120+8)>0; % ADI Hello WorldX
    packetsReceived = uint32(0);
    errors = uint32(0);
end

% Mesg
strAscii = dec2bin('ADI Hello World',8);
msgarray = reshape(strAscii', [1, numel(strAscii)]);
msgbits = logical(msgarray - 48);

% msgLen = uint32(2240);

if valid
    if start
        count = uint32(1);
        packetsReceived = packetsReceived + 1;
    end

    if count <= (length(msgbuffer) - 8)
        msgbuffer(count) = datain;
        if datain ~= msgbits(count)
            errors = errors + 1;
        end

    elseif count == length(msgbuffer) + 1
        msgarray_dec = char('0' + msgbuffer);
        N = length(msgarray_dec) / 8;
        strAscii_dec = reshape(msgarray_dec , 8, N).';
        msg = char(bin2dec(strAscii_dec).');
        disp(msg);
    end
    
    if count <= length(msgbuffer) + 2
        count = count + 1;
    end
end

count_out = count;
packets_out = packetsReceived;
bit_errors_out = errors;

== matlab function commhdlQPSKTxRx/Receiver/QPSK Rx/Frequency and Time Synchronizer/Preamble Detector/FIFO/Validate Input Push Pop/MATLAB Function ==
  data: rst input; count output; enb input; dir input; initVal parameter; countToVal parameter
function count = hdlCounter(rst,enb,dir,initVal,countToVal)
%#codegen

persistent countReg

if(isempty(countReg))
    countReg = fi(initVal,0,nextpow2(countToVal+1),0);
end

if(rst)
    countReg(:) = initVal;
elseif(enb)
    if(dir)
        if(countReg==countToVal)
            countReg(:) = initVal;
        else
            countReg(:) = countReg+1;
        end
    else
        if(countReg==initVal)
            countReg(:) = countToVal;
        else
            countReg(:) = countReg-1;
        end
    end
end

count = countReg;

end

== matlab function commhdlQPSKTxRx/Receiver/QPSK Rx/Frequency and Time Synchronizer/Preamble Detector/FIFO/Validate Input Push Pop/No HDL/MATLAB Function ==
  data: pushFullDiag input; popEmptyDiag input; pushFull input; popEmpty input
function pushPopDiagnostics(pushFullDiag, popEmptyDiag, pushFull, popEmpty)
%#codegen


if(pushFull)
    switch pushFullDiag
        case 2
            warning('Push signal applied on full FIFO');
        case 3
            error('Push signal applied on full FIFO');
        otherwise
    end
end

if(popEmpty)
    switch popEmptyDiag
        case 2
            warning('Pop signal applied on empty FIFO');
        case 3
            error('Pop signal applied on empty FIFO');
        otherwise
    end
end

end

== matlab function commhdlQPSKTxRx/Transmitter/QPSK Tx/Bit Packetizer/Data Bits FIFO/No HDL/MATLAB Function ==
  data: wr input; full output; rd input; ncount output; empty output; dataBitsPerPacket parameter
function [full,ncount,empty] = fcn(wr,rd,dataBitsPerPacket)
%#codegen
     
    depth = dataBitsPerPacket*2 - 1;
    persistent count;
    if isempty(count)
        count = fi(0,0,nextpow2(depth),0,hdlfimath);
    end

    empty = (count == 0);
    full = (count > depth);
    ncount = count;

    if wr
        count(:) = count + 1;
    end
    if rd
        count(:) = count - 1;
    end

end

== matlab function commhdlQPSKTxRx/Receiver/QPSK Rx/Frequency and Time Synchronizer/Packet Controller/MATLAB Function ==
  data: valid input; syncPulse input; out output
function out = fcn(valid,syncPulse)
%#codegen

  persistent Reg;
  if isempty(Reg)
      Reg = false;
  end
  
  out = Reg;
  
  if Reg && valid
      Reg = false;
  end
  
  if syncPulse
      Reg = true;
  end
  
end

== matlab function commhdlQPSKTxRx/Receiver/QPSK Rx/Frequency and Time Synchronizer/Symbol Synchronizer/Rate Handle/FIFO/Validate Input Push Pop/MATLAB Function ==
  data: rst input; count output; enb input; dir input; initVal parameter; countToVal parameter
function count = hdlCounter(rst,enb,dir,initVal,countToVal)
%#codegen

persistent countReg

if(isempty(countReg))
    countReg = fi(initVal,0,nextpow2(countToVal+1),0);
end

if(rst)
    countReg(:) = initVal;
elseif(enb)
    if(dir)
        if(countReg==countToVal)
            countReg(:) = initVal;
        else
            countReg(:) = countReg+1;
        end
    else
        if(countReg==initVal)
            countReg(:) = countToVal;
        else
            countReg(:) = countReg-1;
        end
    end
end

count = countReg;

end

== matlab function commhdlQPSKTxRx/Transmitter/QPSK Tx/Bit Packetizer/Data Bits FIFO/MATLAB Function1 ==
  data: wr input; full output; rd input; dataBitsPerPacket parameter
function full = fcn(wr,rd,dataBitsPerPacket)
%#codegen
     
    depth = dataBitsPerPacket*2 - 1;
    persistent count;
    if isempty(count)
        count = fi(0,0,nextpow2(depth),0,hdlfimath);
    end

    if wr
        count(:) = count + 1;
    end
    if rd
        count(:) = count - 1;
    end

    full = (count > depth);

end

== matlab function commhdlQPSKTxRx/Transmitter/QPSK Tx/Bit Packetizer/Data Bits FIFO/RAM Frame Status Indicator ==
  data: push input; out output; pop input; dataBitsPerPacket parameter
function out = fcn(push,pop,dataBitsPerPacket)

   persistent pushCount popCount frameCount;
   if isempty(pushCount)
       pushCount = fi(0,0,nextpow2(dataBitsPerPacket),0,hdlfimath);
       frameCount = fi(0,0,2,0,hdlfimath);
       popCount = fi(0,0,nextpow2(dataBitsPerPacket),0,hdlfimath);
   end
   
   if (pushCount == dataBitsPerPacket-1) && push
       frameCount(:) = frameCount + 1;
   end
   if (popCount == dataBitsPerPacket-1) && pop
       frameCount(:) = frameCount - 1;
   end

   if push
       if pushCount == dataBitsPerPacket - 1
           pushCount(:) = 0;
       else
           pushCount(:) = pushCount + 1;
       end
   end

   if pop 
       if popCount == dataBitsPerPacket - 1
           popCount(:) = 0;
       else
           popCount(:) = popCount + 1;
       end
   end

   out = frameCount;

end
